simulink model "rs_tlcd_angle_ai"  (R2026a)
settings: Solver=FixedStepDiscrete  StopTime=SIM_TEND  FixedStep=SIM_DT
undefined symbols (not defined in the file or in its folder): POLICY, SIM_DT
settings Model: Creator=cys  LastModifiedBy=cys

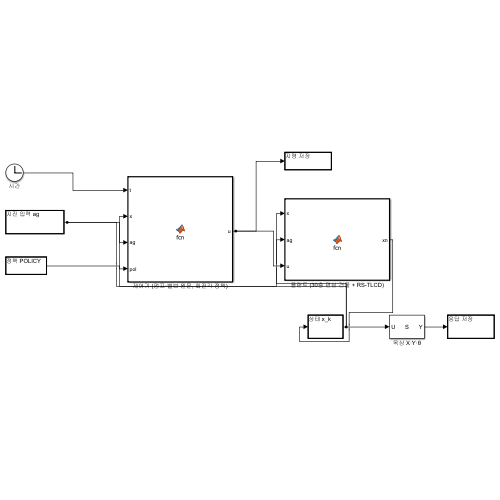
[thumbnail: Simulink's stored preview of the top-level diagram]
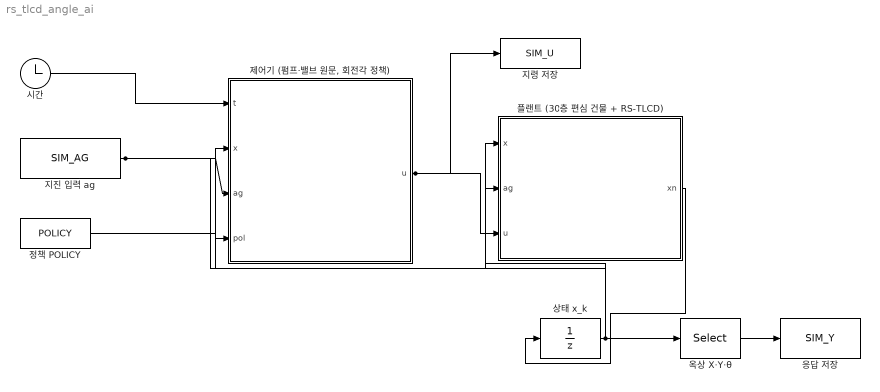
== system rs_tlcd_angle_ai ==
  상태 x_k : UnitDelay  InitialCondition=zeros(184,1)  SampleTime=SIM_DT
  시간 : Clock
  옥상 X·Y·θ : Selector  InputPortWidth=184  IndexOptions=Index vector (dialog)  Indices=[30 61 92]  OutputSizes=1
  응답 저장 : ToWorkspace  VariableName=SIM_Y  SampleTime=SIM_DT
  정책 POLICY : Constant  Value=POLICY  SampleTime=SIM_DT
  "제어기 (펌프·밸브 원문, 회전각 정책)" : MATLAB Function  TreatAsAtomicUnit=on
  지령 저장 : ToWorkspace  VariableName=SIM_U  SampleTime=SIM_DT
  지진 입력 ag : FromWorkspace  VariableName=SIM_AG  SampleTime=SIM_DT  Interpolate=off  OutputAfterFinalValue=Holding final value
  플랜트 (30층 편심 건물 + RS-TLCD) : MATLAB Function  TreatAsAtomicUnit=on
  wires:
  시간/1 -> "제어기 (펌프·밸브 원문, 회전각 정책)"/1(t)
  상태 x_k/1 -> "제어기 (펌프·밸브 원문, 회전각 정책)"/2(x), 플랜트 (30층 편심 건물 + RS-TLCD)/1(x), 옥상 X·Y·θ/1
  지진 입력 ag/1 -> "제어기 (펌프·밸브 원문, 회전각 정책)"/3(ag), 플랜트 (30층 편심 건물 + RS-TLCD)/2(ag)
  정책 POLICY/1 -> "제어기 (펌프·밸브 원문, 회전각 정책)"/4(pol)
  "제어기 (펌프·밸브 원문, 회전각 정책)"/1(u) -> 플랜트 (30층 편심 건물 + RS-TLCD)/3(u), 지령 저장/1
  플랜트 (30층 편심 건물 + RS-TLCD)/1(xn) -> 상태 x_k/1
  옥상 X·Y·θ/1 -> 응답 저장/1

== matlab function rs_tlcd_angle_ai/플랜트 (30층 편심 건물 + RS-TLCD) ==
  data: x input; ag input; u input; xn output
function xn = plant(x, ag, u)
% 이산 상태공간: x_{k+1} = Ad(f,θ) x_k + Bd [ag; F_TLCD]
coder.extrinsic('sim_plant_step');
xn = zeros(184,1);
xn = sim_plant_step(x, ag, u);

== matlab function rs_tlcd_angle_ai/제어기 (펌프·밸브 원문, 회전각 정책) ==
  data: t input; u output; x input; ag input; pol input
function u = ctrl(t, x, ag, pol)
% 원문 펌프(식 10·11)·밸브(식 12)·회전 속도 제한 + 회전 목표각 정책
coder.extrinsic('sim_ctrl_step');
u = zeros(4,1);
u = sim_ctrl_step(t, x, ag, pol);
